simulink library "ndi_lib"  (R2018b)
settings: Solver=VariableStepAuto  StartTime=0.0  StopTime=10.0  RelTol=1e-3
undefined symbols (not defined in the file or in its folder): cntrl
libraries: filters_lib x4
settings Model: Creator=Ybeyer  LastModifiedBy=yannic
settings DebuggingCC: LibraryContextMissingDiagnostic=none
settings SFSimCC: SimUseLocalCustomCode=off
settings RTWCC: RTWUseLocalCustomCode=off
settings CodeAppCC: StateflowObjectComments=on

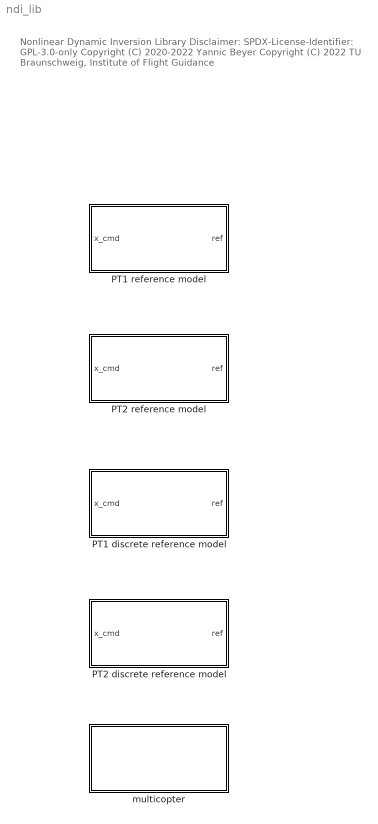
== system ndi_lib ==
  note: Nonlinear Dynamic Inversion Library
      |
      | Disclaimer:
      | SPDX-License-Identifier: GPL-3.0-only
      |
      | Copyright (C) 2020-2022 Yannic Beyer
      | Copyright (C) 2022 TU Braunschweig, Institute of Flight Guidance
  PT1 discrete reference model : Subsystem  mask{T=1, x_max=inf, x_min=-inf, x_dt_max=inf, x_dt_min=-inf, x_init=0}
      mask prompts: T "Time constant"; x_max "Maximum position"; x_min "Minimum position"; x_dt_max "Maximum rate"; x_dt_min "Minimum rate"; x_init "Initial position"
  PT1 reference model : Subsystem  mask{T=1, x_max=inf, x_min=-inf, x_dt_max=inf, x_dt_min=-inf, x_init=0}
      mask prompts: T "Time constant"; x_max "Maximum position"; x_min "Minimum position"; x_dt_max "Maximum rate"; x_dt_min "Minimum rate"; x_init "Initial position"
  PT2 discrete reference model : Subsystem  mask{omega=[cntrl.rm.Phi.omega], d=[cntrl.rm.Phi.D], x_dt2_max=inf, x_dt2_min=-inf, x_dt_max=inf, x_dt_min=-inf, x_max=inf, x_min=-inf, x_init=[1;0;0;0], x_dt_init=0}
      mask prompts: omega "Natural frequency"; d "Damping ratio"; x_dt2_max "Maximum acceleration"; x_dt2_min "Minimum acceleration"; x_dt_max "Maximum rate"; x_dt_min "Minimum rate"; x_max "Maximum position"; x_min "Minimum position"; x_init "Initial position"; x_dt_init "Initial rate"
  PT2 reference model : Subsystem  mask{omega=0.7, d=1, x_dt2_max=inf, x_dt2_min=-inf, x_dt_max=inf, x_dt_min=-inf, x_max=inf, x_min=-inf, x_init=0, x_dt_init=0}
      mask prompts: omega "Natural frequency"; d "Damping ratio"; x_dt2_max "Maximum acceleration"; x_dt2_min "Minimum acceleration"; x_dt_max "Maximum rate"; x_dt_min "Minimum rate"; x_max "Maximum position"; x_min "Minimum position"; x_init "Initial position"; x_dt_init "Initial rate"
  multicopter : Subsystem
      settings: OpenFcn=multicopterNDI_lib

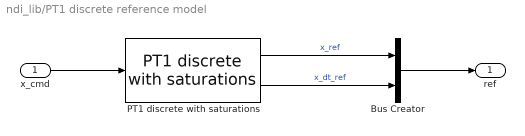
== system ndi_lib/PT1 discrete reference model ==
  x_cmd : Inport
  Bus Creator : BusCreator  Inputs=2
  PT1 discrete with saturations : filters_lib/PT1 discrete with saturations  T=T  x_max=x_max  x_min=x_min  x_dt_max=x_dt_max  x_dt_min=x_dt_min  x_init=x_init
      settings: SourceProductName=LADAC
  ref : Outport
  wires:
  PT1 discrete with saturations/2 -> Bus Creator/2  "x_dt_ref"
  PT1 discrete with saturations/1 -> Bus Creator/1  "x_ref"
  Bus Creator/1 -> ref/1
  x_cmd/1 -> PT1 discrete with saturations/1

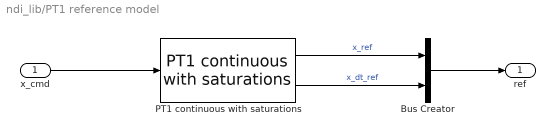
== system ndi_lib/PT1 reference model ==
  x_cmd : Inport
  Bus Creator : BusCreator  Inputs=2
  PT1 continuous with saturations : filters_lib/PT1 continuous with saturations  T=T  x_max=x_max  x_min=x_min  x_dt_max=x_dt_max  x_dt_min=x_dt_min  x_init=x_init
      settings: SourceProductName=LADAC
  ref : Outport
  wires:
  PT1 continuous with saturations/2 -> Bus Creator/2  "x_dt_ref"
  PT1 continuous with saturations/1 -> Bus Creator/1  "x_ref"
  Bus Creator/1 -> ref/1
  x_cmd/1 -> PT1 continuous with saturations/1

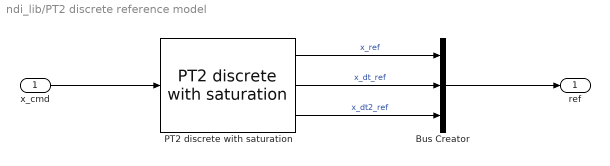
== system ndi_lib/PT2 discrete reference model ==
  x_cmd : Inport
  Bus Creator : BusCreator  Inputs=3
  PT2 discrete with saturation : filters_lib/PT2 discrete with saturation  omega=omega  d=d  x_dt2_max=x_dt2_max  x_dt2_min=x_dt2_min  x_dt_max=x_dt_max  x_dt_min=x_dt_min  x_max=x_max  x_min=x_min  x_init=x_init  x_dt_init=x_dt_init
      settings: SourceProductName=LADAC
  ref : Outport
  wires:
  PT2 discrete with saturation/3 -> Bus Creator/3  "x_dt2_ref"
  Bus Creator/1 -> ref/1
  PT2 discrete with saturation/1 -> Bus Creator/1  "x_ref"
  PT2 discrete with saturation/2 -> Bus Creator/2  "x_dt_ref"
  x_cmd/1 -> PT2 discrete with saturation/1

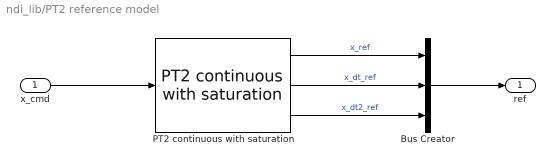
== system ndi_lib/PT2 reference model ==
  x_cmd : Inport
  Bus Creator : BusCreator  Inputs=3
  PT2 continuous with saturation : filters_lib/PT2 continuous with saturation  omega=omega  d=d  x_dt2_max=x_dt2_max  x_dt2_min=x_dt2_min  x_dt_max=x_dt_max  x_dt_min=x_dt_min  x_max=x_max  x_min=x_min  x_init=x_init  x_dt_init=x_dt_init
      settings: SourceProductName=LADAC
  ref : Outport
  wires:
  PT2 continuous with saturation/2 -> Bus Creator/2  "x_dt_ref"
  PT2 continuous with saturation/1 -> Bus Creator/1  "x_ref"
  Bus Creator/1 -> ref/1
  PT2 continuous with saturation/3 -> Bus Creator/3  "x_dt2_ref"
  x_cmd/1 -> PT2 continuous with saturation/1

== system ndi_lib/multicopter ==
